simulink model "separately_excited_dc_generator"  (R2023b)
settings: Solver=VariableStepAuto  StartTime=0.0  StopTime=10.0  RelTol=1e-3
libraries: spsDCVoltageSourceLib x2, spsDCMachineLib x1, sps_lib x1
settings Model: Creator=Yunus Emre Turunç  LastModifiedBy=Yunus Emre Turunç

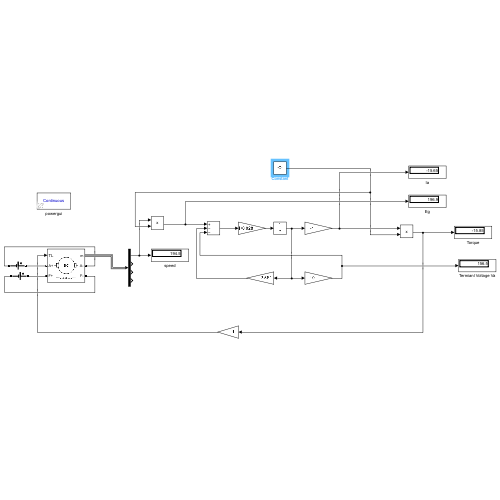
[thumbnail: Simulink's stored preview of the top-level diagram]
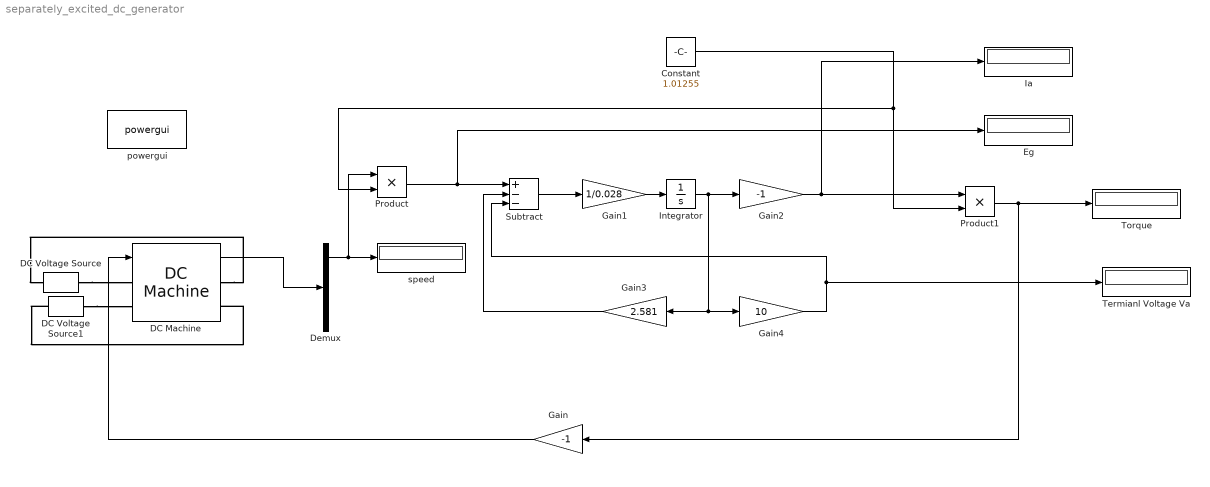
== system separately_excited_dc_generator ==
  Constant : Constant  Value=1.01255
  DC Machine : spsDCMachineLib/DC Machine  PresetModel=01: 5HP 240V 1750RPM Field:300V  MechanicalLoad=Torque TL  FieldType=Wound  ShowDetailedParameters=on  MeasurementBus=off  RLa=[2.581 0.028]  RLf=[281.2 156]  Laf=0.9483  MachineConstant=Torque constant (N.m/A)  Ke=1.8  Kt=1.8  J=0.02215  Bm=0.002953  Tf=0.5161  w0=1  Ifinit=1.06685633001422  TsPowergui=0  TsBlock=-1
  DC Voltage Source : spsDCVoltageSourceLib/DC Voltage Source  Amplitude=240  Measurements=None
  DC Voltage Source1 : spsDCVoltageSourceLib/DC Voltage Source  Amplitude=300  Measurements=None
  Demux : Demux
  Eg : Display
  Gain : Gain  Gain=-1
  Gain1 : Gain  Gain=1/0.028
  Gain2 : Gain  Gain=-1
  Gain3 : Gain  Gain=2.581
  Gain4 : Gain  Gain=10
  Ia : Display
  Integrator : Integrator
  Product : Product
  Product1 : Product
  Subtract : Sum  Inputs=+--
  Termianl Voltage Va : Display
  Torque : Display
  powergui : sps_lib/powergui  Priority=1  SimulationMode=Continuous  SampleTime=50e-6  frequency=60  Iterations=50  frequencyindice=0  Pbase=100e6  ErrMax=1e-4  UnitsV=kV  UnitsW=MW  buscounter=0  FunctionMessages=off  echomessages=off  EnableUseOfTLC=off  CurrentSourceSwitches=off  DisableSnubberDevices=off  DisableRonSwitches=off  DisableVfSwitches=off  DisplayEquations=off  AutomaticDiscreteSolvers=off  SolverType=Tustin/Backward Euler (TBE)  Interpol=off  ExternalGateDelay=off  methode=off  Ts=100  x0status=blocks  SPID=on  SwTol=0  HookPort=off  NonlinearTolerance=1e-4  nMaxIteration=100  ContinueOnMaxIteration=off  RestoreLinks=warning  ResistiveCurrentMeasurement=off  Frange=[0:2:500]  Ylog=off  Xlog=on  ShowGrid=off  save=off  variable=ZData  structure=0  ZoomFFT=off  StartTime=0.0  cycles=1  DisplayStyle=1  fundamental=60  FreqAxis=off  MaxFrequency=1000  frequencyindicesteady=1  RmsSteady=1  display=off
  speed : Display
  wires:
  DC Machine/1 -> Demux/1
  Demux/1 -> Product/1, speed/1
  Gain/1 -> DC Machine/1
  Product/1 -> Eg/1, Subtract/1
  Subtract/1 -> Gain1/1
  Gain1/1 -> Integrator/1
  Gain2/1 -> Ia/1, Product1/1
  Constant/1 -> Product/2, Product1/2
  Integrator/1 -> Gain4/1, Gain3/1, Gain2/1
  Gain3/1 -> Subtract/2
  Gain4/1 -> Subtract/3, Termianl Voltage Va/1
  Product1/1 -> Torque/1, Gain/1
  connections:
  DC Voltage Source/RConn1 -- DC Machine/LConn1
  DC Voltage Source1/RConn1 -- DC Machine/LConn2
  DC Machine/RConn1 -- DC Voltage Source/LConn1
  DC Voltage Source1/LConn1 -- DC Machine/RConn2
